simulink model "MMC_phase_discentralized_HAAS_20260927"  (R2024b)
settings: Solver=FixedStepDiscrete  StartTime=t_init_sim  StopTime=sim_time  FixedStep=Ts  RelTol=1e-3
values from neighbouring files (symbols this model uses):
  a = 1    [script_MMC_phase_hackathon_NLM_discentralized_HAAS_20260927.m]
  C1low1_active = 1    [script_MMC_phase_hackathon_NLM_discentralized_HAAS_20260927.m]
  C2low1_active = 1    [script_MMC_phase_hackathon_NLM_discentralized_HAAS_20260927.m]
  C_bus = 4400e-6    (= 0.0044)    [script_MMC_phase_hackathon_NLM_discentralized_HAAS_20260927.m]
  C_M_extra = C_m-twist_high_side_C    [script_MMC_phase_hackathon_NLM_discentralized_HAAS_20260927.m]
  duty_cycle = 1.0    (= 1)    [script_MMC_phase_hackathon_NLM_discentralized_HAAS_20260927.m]
  f0 = 50    [script_MMC_phase_hackathon_NLM_discentralized_HAAS_20260927.m]
  feeder_current_lower_rate_limit = -10    [script_MMC_phase_hackathon_NLM_discentralized_HAAS_20260927.m]    (also in twist_parameters.m = -500)
  feeder_current_tab = [0.328 0.217 0.162 0.132 0.109 0.094 0.083 0.075 0.068 0.062 0.058 0.054 ... (42 elements, 14x3)]    [feeder_current.mat]
  feeder_current_upper_rate_limit = 0.386/(20e-3)    (= 19.3)    [twist_parameters.m]
  is6VExternallySupplied = true    [script_MMC_phase_hackathon_NLM_discentralized_HAAS_20260927.m]
  isFeederJumperOpen = true    [script_MMC_phase_hackathon_NLM_discentralized_HAAS_20260927.m]
  L_arm = 30e-3    (= 0.03)    [script_MMC_phase_hackathon_NLM_discentralized_HAAS_20260927.m]
  m = 1    [script_MMC_phase_hackathon_NLM_discentralized_HAAS_20260927.m]
  N = 5    [script_MMC_phase_hackathon_NLM_discentralized_HAAS_20260927.m]
  power_losses = false    [script_MMC_phase_hackathon_NLM_discentralized_HAAS_20260927.m]
  R = 15    [script_MMC_phase_hackathon_NLM_discentralized_HAAS_20260927.m]
  R_arm = 0.2    [script_MMC_phase_hackathon_NLM_discentralized_HAAS_20260927.m]
  source_V = 0    [script_MMC_phase_hackathon_NLM_discentralized_HAAS_20260927.m]
  Tcom_sample = round(Tcom / Ts)    [script_MMC_phase_hackathon_NLM_discentralized_HAAS_20260927.m]
  time_charge = 0.1    [script_MMC_phase_hackathon_NLM_discentralized_HAAS_20260927.m]
  time_decharge = 1.5    [script_MMC_phase_hackathon_NLM_discentralized_HAAS_20260927.m]
  Ts = 1e-6    (= 1e-06)    [script_MMC_phase_hackathon_NLM_discentralized_HAAS_20260927.m]
  twist_data_acquisition_delay = 50e-9    (= 5e-08)    [script_MMC_phase_hackathon_NLM_discentralized_HAAS_20260927.m]    (also in twist_parameters.m)
  twist_data_sampling_period = 1/twist_freq_data_sampling    (= 5e-05)    [script_MMC_phase_hackathon_NLM_discentralized_HAAS_20260927.m]    (also in twist_parameters.m)
  twist_dead_time = 200e-9    (= 2e-07)    [twist_parameters.m]
  twist_freq_switching = 200e3    (= 200000)    [twist_parameters.m]
  twist_high_side_adc_R = 1/(1/2e6 + 1/2e6 + 1/(330e3+5.6e3))    (= 251272.836178)    [twist_parameters.m]
  twist_high_side_C = 33e-6*4 + 4.7e-6*12    (= 0.0001884)    [twist_parameters.m]
  twist_high_side_feeder_R = 47e3+4.7e3    (= 51700)    [twist_parameters.m]
  twist_high_side_rC = 0.1    [twist_parameters.m]
  twist_low_side_adc_R = 150e3+470    (= 150470)    [twist_parameters.m]
  twist_low_side_C_ceramic = 3*4.7e-6    (= 1.41e-05)    [twist_parameters.m]
  twist_low_side_C_electrolytic = 47e-6    (= 4.7e-05)    [twist_parameters.m]
  twist_low_side_L = 33e-6    (= 3.3e-05)    [twist_parameters.m]
  twist_low_side_rC = 700e-3    (= 0.7)    [twist_parameters.m]
  twist_low_side_rL = 20e-3    (= 0.02)    [twist_parameters.m]
  twist_R_VCC = (tau_VCC/twist_high_side_C  - twist_high_side_rC)/(1-(tau_VCC/twist_high_side_C - twist_high_side_rC)/R_parallel)    (= 1110.74997822)    [twist_parameters.m]
  VDC = 48    [script_MMC_phase_hackathon_NLM_discentralized_HAAS_20260927.m]
undefined symbols (not defined in the file or in its folder): C_SM, feeder_current, gcbh, sps_rtmsupport, twist_low_side_lC
libraries: spsSeriesRLCBranchLib x135, spsTriangleGeneratorLib x60, spsMosfetLib x60, spsCurrentMeasurementLib x43, spsVoltageMeasurementLib x35, spsControlledCurrentSourceLib x30, spsDiodeLib x22, spsIdealSwitchLib x20, spsControlledVoltageSourceLib x1, spsGroundLib x1, spspowerguiLib x1
(part 4 of 22)

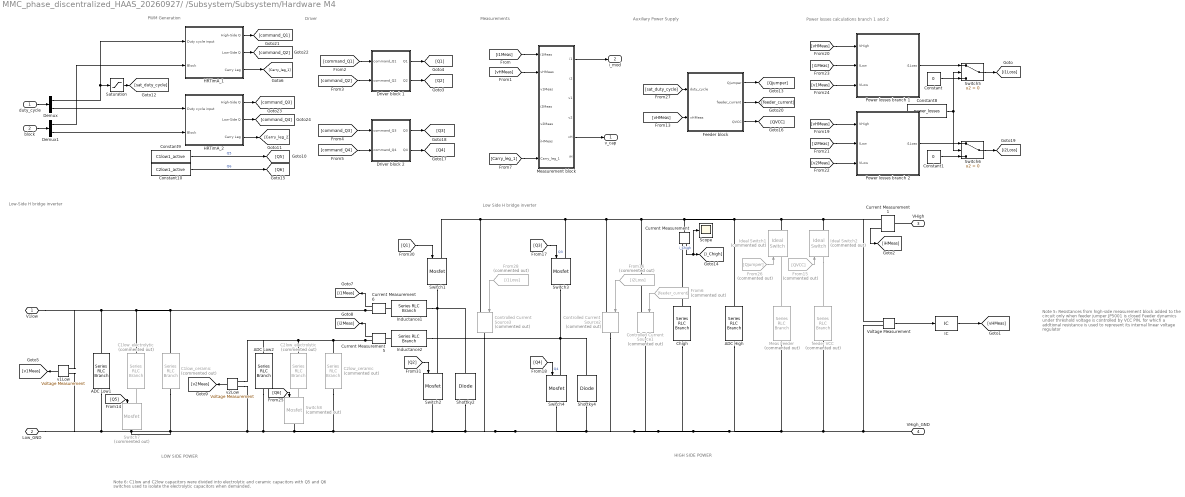
== system MMC_phase_discentralized_HAAS_20260927/ /Subsystem/Subsystem/Hardware M4 ==
  note: Low Side H bridge inverter
  note: PWM Generation
  note: Auxiliary Power Supply
  note: LOW SIDE POWER
  note: Low-Side H bridge inverter
  note: Power losses calculations branch 1 and 2
  note: Note 6:
      | C1low and C2low capacitors were divided into electrolytic and ceramic capacitors with Q5 and Q6 switches used to isolate the electrolytic capacitors when demanded.
  note: HIGH SIDE POWER
  note: Measurements
  note: Note 5:
      |
      | Resistances from high-side measurement block added to the circuit only when feeder jumper JP5001 is closed
      |
      | Feeder dynamics under threshold voltage is controlled by VCC PIN, for which a addtional resistance is used to represent its internal linear voltage regulator
  note: Driver
  duty_cycle : Inport
  block : Inport  Port=2
  ADC High : spsSeriesRLCBranchLib/Series RLC Branch  LConnTagsString=__new0  RConnTagsString=__new0  BranchType=R  Resistance=twist_high_side_adc_R  Inductance=twist_low_side_L  SetiL0=off  InitialCurrent=0  Capacitance=1e-6  Setx0=off  InitialVoltage=0  Measurements=None
  ADC Low1 : spsSeriesRLCBranchLib/Series RLC Branch  LConnTagsString=__new0  RConnTagsString=__new0  BranchType=R  Resistance=twist_low_side_adc_R  Inductance=twist_low_side_L  SetiL0=off  InitialCurrent=0  Capacitance=1e-6  Setx0=off  InitialVoltage=0  Measurements=Branch voltage
  ADC Low2 : spsSeriesRLCBranchLib/Series RLC Branch  LConnTagsString=__new0  RConnTagsString=__new0  BranchType=R  Resistance=twist_low_side_adc_R  Inductance=twist_low_side_L  SetiL0=off  InitialCurrent=0  Capacitance=1e-6  Setx0=off  InitialVoltage=0  Measurements=Branch voltage
  C1low_ceramic : spsSeriesRLCBranchLib/Series RLC Branch  Commented=on  LConnTagsString=__new0  RConnTagsString=__new0  BranchType=C  Resistance=twist_low_side_rC  Inductance=1e-3  SetiL0=off  InitialCurrent=0  Capacitance=twist_low_side_C_ceramic  Setx0=off  InitialVoltage=source_V  Measurements=None
  C1low_electrolytic : spsSeriesRLCBranchLib/Series RLC Branch  Commented=on  LConnTagsString=__new0  RConnTagsString=__new0  BranchType=RC  Resistance=twist_low_side_rC  Inductance=twist_low_side_lC  SetiL0=off  InitialCurrent=0  Capacitance=twist_low_side_C_electrolytic  Setx0=off  InitialVoltage=source_V  Measurements=None
  C2low_ceramic : spsSeriesRLCBranchLib/Series RLC Branch  Commented=on  LConnTagsString=__new0  RConnTagsString=__new0  BranchType=C  Resistance=twist_low_side_rC  Inductance=1e-3  SetiL0=off  InitialCurrent=0  Capacitance=twist_low_side_C_ceramic  Setx0=off  InitialVoltage=source_V  Measurements=None
  C2low_electrolytic : spsSeriesRLCBranchLib/Series RLC Branch  Commented=on  LConnTagsString=__new0  RConnTagsString=__new0  BranchType=RC  Resistance=twist_low_side_rC  Inductance=twist_low_side_lC  SetiL0=off  InitialCurrent=0  Capacitance=twist_low_side_C_electrolytic  Setx0=off  InitialVoltage=source_V  Measurements=None
  Chigh : spsSeriesRLCBranchLib/Series RLC Branch  LConnTagsString=__new0  RConnTagsString=__new0  BranchType=RC  Resistance=twist_high_side_rC  Inductance=1e-3  SetiL0=off  InitialCurrent=0  Capacitance=twist_high_side_C  Setx0=on  InitialVoltage=source_V  Measurements=None
  Constant : Constant  Value=0
  Constant1 : Constant  Value=0
  Constant10 : Constant  Value=C2low1_active
  Constant8 : Constant  Value=power_losses
  Constant9 : Constant  Value=C1low1_active
  Controlled Current Source1 : spsControlledCurrentSourceLib/Controlled Current Source  Commented=on  Initialize=on  Source_Type=AC  Amplitude=0  Phase=0  Frequency=0  Measurements=None
  Controlled Current Source2 : spsControlledCurrentSourceLib/Controlled Current Source  Commented=on  Initialize=on  Source_Type=AC  Amplitude=0  Phase=0  Frequency=0  Measurements=None
  Controlled Current Source3 : spsControlledCurrentSourceLib/Controlled Current Source  Commented=on  Initialize=on  Source_Type=AC  Amplitude=0  Phase=0  Frequency=0  Measurements=None
  Current Measurement{,1,5..6} (4 alike) : spsCurrentMeasurementLib/Current Measurement  PhasorSimulation=off  OutputType=Complex  PSBequivalent=0
  Demux : Demux  Outputs=2
  Demux1 : Demux  Outputs=2
  Driver block 1 : Subsystem
  Driver block 2 : Subsystem
  Feeder block : Subsystem
  From15 : From  Commented=on  GotoTag=QVCC
  From16 : From  Commented=on  GotoTag=i2Loss
  From26 : From  Commented=on  GotoTag=Qjumper
  From28 : From  Commented=on  GotoTag=i1Loss
  From6 : From  Commented=on  GotoTag=feeder_current
  HRTimA_1 : Subsystem
  HRTimA_2 : Subsystem
  IC : InitialCondition  Value=source_V
  Ideal Switch1 : spsIdealSwitchLib/Ideal Switch  Commented=on  Ron=0.001  Lon=0  IC=0  Rs=1e5  Cs=inf  Measurements=on
  Ideal Switch2 : spsIdealSwitchLib/Ideal Switch  Commented=on  Ron=0.001  Lon=0  IC=0  Rs=1e5  Cs=inf  Measurements=on
  Inductance1 : spsSeriesRLCBranchLib/Series RLC Branch  LConnTagsString=__new0  RConnTagsString=__new0  BranchType=RL  Resistance=twist_low_side_rL  Inductance=twist_low_side_L  SetiL0=off  InitialCurrent=0  Capacitance=1e-6  Setx0=off  InitialVoltage=0  Measurements=None
  Inductance2 : spsSeriesRLCBranchLib/Series RLC Branch  LConnTagsString=__new0  RConnTagsString=__new0  BranchType=RL  Resistance=twist_low_side_rL  Inductance=twist_low_side_L  SetiL0=off  InitialCurrent=0  Capacitance=1e-6  Setx0=off  InitialVoltage=0  Measurements=None
  Meas Feeder : spsSeriesRLCBranchLib/Series RLC Branch  Commented=on  LConnTagsString=__new0  RConnTagsString=__new0  BranchType=R  Resistance=twist_high_side_feeder_R  Inductance=twist_low_side_L  SetiL0=off  InitialCurrent=0  Capacitance=1e-6  Setx0=off  InitialVoltage=0  Measurements=None
  Measurement block : Subsystem
  Power losses branch 1 : Subsystem
  Power losses branch 2 : Subsystem
  Saturation : Saturate  UpperLimit=1  LowerLimit=0
  Scope : Scope
  Shottky2 : spsDiodeLib/Diode  Ron=twist_shottky_Ron  Lon=0  Vf=twist_shottky_Vf  IC=0  UseSnubber=0  Rs=twist_shottky_Rs  Cs=twist_shottky_Cs  Measurements=off
  Shottky4 : spsDiodeLib/Diode  Ron=twist_shottky_Ron  Lon=0  Vf=twist_shottky_Vf  IC=0  UseSnubber=0  Rs=twist_shottky_Rs  Cs=twist_shottky_Cs  Measurements=off
  Switch{1..4} (4 alike) : spsMosfetLib/Mosfet  Ron=twist_FET_Ron  Lon=0  Rd=twist_FET_Rd  Vfd=twist_FET_Vf  IC=0  Rs=twist_FET_Rs  Cs=twist_FET_Cs  Measurements=off
  Switch5 : Switch  Criteria=u2 > Threshold  SaturateOnIntegerOverflow=off  InputSameDT=off
  Switch6 : Switch  Criteria=u2 > Threshold  SaturateOnIntegerOverflow=off  InputSameDT=off
  Switch7 : spsMosfetLib/Mosfet  Commented=on  Ron=twist_FET_Clow_Ron  Lon=0  Rd=twist_FET_Clow_Ron  Vfd=0  IC=0  Rs=twist_FET_Rs  Cs=twist_FET_Cs  Measurements=off
  Switch8 : spsMosfetLib/Mosfet  Commented=on  Ron=twist_FET_Clow_Ron  Lon=0  Rd=twist_FET_Clow_Ron  Vfd=0  IC=0  Rs=twist_FET_Rs  Cs=twist_FET_Cs  Measurements=off
  Voltage Measurement : spsVoltageMeasurementLib/Voltage Measurement  PhasorSimulation=off  OutputType=Complex  PSBequivalent=0
  feeder VCC : spsSeriesRLCBranchLib/Series RLC Branch  Commented=on  LConnTagsString=__new0  RConnTagsString=__new0  BranchType=R  Resistance=twist_R_VCC  Inductance=twist_low_side_L  SetiL0=off  InitialCurrent=0  Capacitance=1e-6  Setx0=off  InitialVoltage=0  Measurements=None
  v1Low : spsVoltageMeasurementLib/Voltage Measurement  PhasorSimulation=off  OutputType=Complex  PSBequivalent=0
  v2Low : spsVoltageMeasurementLib/Voltage Measurement  PhasorSimulation=off  OutputType=Complex  PSBequivalent=0
  V1low : PMIOPort  Side=Left
  Low_GND : PMIOPort  Port=2  Side=Left
  VHigh : PMIOPort  Port=3  Side=Right
  VHigh_GND : PMIOPort  Port=4  Side=Right
  v_cap : Outport
  i_mod : Outport  Port=2
  wires:
  Constant8/1 -> Switch5/2, Switch6/2
  Constant9/1 -> [Q5]  "Q5"
  Constant1/1 -> Switch6/3
  v1Low/1 -> [v1Meas]
  Power losses branch 1/1(i1Loss) -> Switch5/1
  Constant/1 -> Switch5/3
  [Q1] -> Switch1/1
  [Q3] -> Switch3/1  "Q3"
  Voltage Measurement/1 -> IC/1
  Constant10/1 -> [Q6]  "Q6"
  [v1Meas] -> Power losses branch 1/3(VLow)
  [i2Meas] -> Power losses branch 2/2(ILow)
  Switch5/1 -> [i1Loss]
  HRTimA_2/3(Carry Leg) -> [Carry_leg_2]
  Current Measurement1/1 -> [iHMeas]
  v2Low/1 -> [v2Meas]
  HRTimA_1/3(Carry Leg) -> [Carry_leg_1]
  [vHMeas] -> Power losses branch 1/1(VHigh)
  IC/1 -> [vHMeas]
  From28/1 -> Controlled Current Source3/1
  Current Measurement/1 -> Scope/1, [i_Chigh]  "i_Chigh"
  Switch6/1 -> [i2Loss]
  Current Measurement5/1 -> [i2Meas]
  From26/1 -> Ideal Switch1/1
  [i1Meas] -> Power losses branch 1/2(ILow)
  From15/1 -> Ideal Switch2/1
  [Q5] -> Switch7/1
  [Q6] -> Switch8/1
  [Q4] -> Switch4/1  "Q4"
  [Q2] -> Switch2/1
  From6/1 -> Controlled Current Source1/1
  [vHMeas] -> Power losses branch 2/1(VHigh)
  From16/1 -> Controlled Current Source2/1
  [v2Meas] -> Power losses branch 2/3(VLow)
  Current Measurement6/1 -> [i1Meas]
  Power losses branch 2/1(i1Loss) -> Switch6/1
  duty_cycle/1 -> Demux/1
  Demux/1 -> Saturation/1, HRTimA_1/1(Duty cycle input)
  Demux1/1 -> HRTimA_1/2(Block)
  block/1 -> Demux1/1
  Demux1/2 -> HRTimA_2/2(Block)
  Demux/2 -> HRTimA_2/1(Duty cycle input)
  [vHMeas] -> Feeder block/2(vHMeas)
  Saturation/1 -> [sat_duty_cycle]
  [sat_duty_cycle] -> Feeder block/1(duty_cycle)
  Feeder block/1(Qjumper) -> [Qjumper]
  Feeder block/3(QVCC) -> [QVCC]
  Feeder block/2(feeder_current) -> [feeder_current]
  Measurement block/1(i1) -> i_mod/1
  [i1Meas] -> Measurement block/1(i1Meas)
  [vHMeas] -> Measurement block/2(vHMeas)
  Measurement block/5(vH) -> v_cap/1
  HRTimA_1/1(High-Side Q) -> [command_Q1]
  HRTimA_1/2(Low-Side Q) -> [command_Q2]
  HRTimA_2/1(High-Side Q) -> [command_Q3]
  HRTimA_2/2(Low-Side Q) -> [command_Q4]
  [command_Q1] -> Driver block 1/1(command_Q1)
  [command_Q2] -> Driver block 1/2(command_Q2)
  [command_Q3] -> Driver block 2/1(command_Q3)
  [command_Q4] -> Driver block 2/2(command_Q4)
  Driver block 1/1(Q1) -> [Q1]
  Driver block 1/2(Q2) -> [Q2]
  Driver block 2/1(Q3) -> [Q3]
  Driver block 2/2(Q4) -> [Q4]
  [Carry_leg_1] -> Measurement block/7(Carry_leg_1)
  connections:
  Current Measurement6/RConn1 -- v1Low/LConn1 -- V1low/RConn1 -- ADC Low1/LConn1 -- C1low_electrolytic/LConn1 -- C1low_ceramic/LConn1
  Switch3/LConn1 -- Controlled Current Source3/LConn1 -- Switch1/LConn1 -- Current Measurement/LConn1 -- Ideal Switch1/RConn1 -- Voltage Measurement/LConn1 -- Current Measurement1/RConn1 -- Ideal Switch2/RConn1 -- ADC High/LConn1 -- Controlled Current Source1/LConn1 -- Controlled Current Source2/LConn1
  VHigh_GND/RConn1 -- Voltage Measurement/LConn2 -- feeder VCC/RConn1 -- ADC High/RConn1 -- Chigh/RConn1 -- Controlled Current Source2/RConn1 -- Controlled Current Source3/RConn1 -- Switch2/RConn1 -- Low_GND/RConn1 -- v1Low/LConn2 -- ADC Low1/RConn1 -- Switch7/RConn1 -- C1low_ceramic/RConn1 -- v2Low/LConn2 -- ADC Low2/RConn1 -- Switch8/RConn1 -- C2low_ceramic/RConn1 -- Shottky2/LConn1 -- Switch4/RConn1 -- Shottky4/LConn1 -- Controlled Current Source1/RConn1 -- Meas Feeder/RConn1
  Current Measurement5/RConn1 -- v2Low/LConn1 -- ADC Low2/LConn1 -- C2low_electrolytic/LConn1 -- C2low_ceramic/LConn1
  Inductance2/RConn1 -- Switch4/LConn1 -- Switch3/RConn1 -- Shottky4/RConn1
  Switch1/RConn1 -- Inductance1/RConn1 -- Shottky2/RConn1 -- Switch2/LConn1
  Meas Feeder/LConn1 -- Ideal Switch1/LConn1
  Inductance2/LConn1 -- Current Measurement5/LConn1
  Switch7/LConn1 -- C1low_electrolytic/RConn1
  Ideal Switch2/LConn1 -- feeder VCC/LConn1
  Switch8/LConn1 -- C2low_electrolytic/RConn1
  Current Measurement/RConn1 -- Chigh/LConn1
  VHigh/RConn1 -- Current Measurement1/LConn1
  Current Measurement6/LConn1 -- Inductance1/LConn1

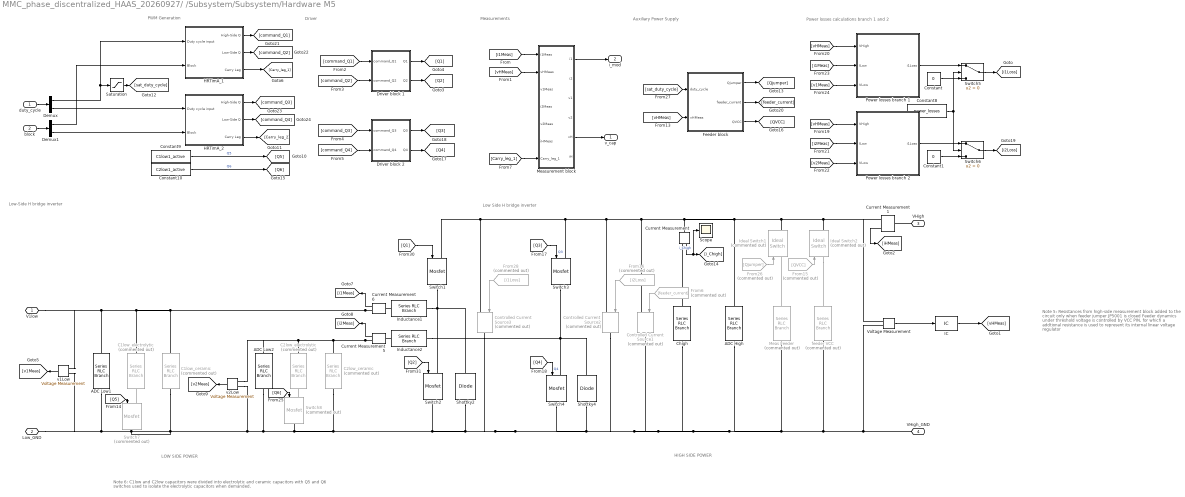
== system MMC_phase_discentralized_HAAS_20260927/ /Subsystem/Subsystem/Hardware M5 ==
  note: Low Side H bridge inverter
  note: PWM Generation
  note: Auxiliary Power Supply
  note: LOW SIDE POWER
  note: Low-Side H bridge inverter
  note: Power losses calculations branch 1 and 2
  note: Note 6:
      | C1low and C2low capacitors were divided into electrolytic and ceramic capacitors with Q5 and Q6 switches used to isolate the electrolytic capacitors when demanded.
  note: HIGH SIDE POWER
  note: Measurements
  note: Note 5:
      |
      | Resistances from high-side measurement block added to the circuit only when feeder jumper JP5001 is closed
      |
      | Feeder dynamics under threshold voltage is controlled by VCC PIN, for which a addtional resistance is used to represent its internal linear voltage regulator
  note: Driver
  duty_cycle : Inport
  block : Inport  Port=2
  ADC High : spsSeriesRLCBranchLib/Series RLC Branch  LConnTagsString=__new0  RConnTagsString=__new0  BranchType=R  Resistance=twist_high_side_adc_R  Inductance=twist_low_side_L  SetiL0=off  InitialCurrent=0  Capacitance=1e-6  Setx0=off  InitialVoltage=0  Measurements=None
  ADC Low1 : spsSeriesRLCBranchLib/Series RLC Branch  LConnTagsString=__new0  RConnTagsString=__new0  BranchType=R  Resistance=twist_low_side_adc_R  Inductance=twist_low_side_L  SetiL0=off  InitialCurrent=0  Capacitance=1e-6  Setx0=off  InitialVoltage=0  Measurements=Branch voltage
  ADC Low2 : spsSeriesRLCBranchLib/Series RLC Branch  LConnTagsString=__new0  RConnTagsString=__new0  BranchType=R  Resistance=twist_low_side_adc_R  Inductance=twist_low_side_L  SetiL0=off  InitialCurrent=0  Capacitance=1e-6  Setx0=off  InitialVoltage=0  Measurements=Branch voltage
  C1low_ceramic : spsSeriesRLCBranchLib/Series RLC Branch  Commented=on  LConnTagsString=__new0  RConnTagsString=__new0  BranchType=C  Resistance=twist_low_side_rC  Inductance=1e-3  SetiL0=off  InitialCurrent=0  Capacitance=twist_low_side_C_ceramic  Setx0=off  InitialVoltage=source_V  Measurements=None
  C1low_electrolytic : spsSeriesRLCBranchLib/Series RLC Branch  Commented=on  LConnTagsString=__new0  RConnTagsString=__new0  BranchType=RC  Resistance=twist_low_side_rC  Inductance=twist_low_side_lC  SetiL0=off  InitialCurrent=0  Capacitance=twist_low_side_C_electrolytic  Setx0=off  InitialVoltage=source_V  Measurements=None
  C2low_ceramic : spsSeriesRLCBranchLib/Series RLC Branch  Commented=on  LConnTagsString=__new0  RConnTagsString=__new0  BranchType=C  Resistance=twist_low_side_rC  Inductance=1e-3  SetiL0=off  InitialCurrent=0  Capacitance=twist_low_side_C_ceramic  Setx0=off  InitialVoltage=source_V  Measurements=None
  C2low_electrolytic : spsSeriesRLCBranchLib/Series RLC Branch  Commented=on  LConnTagsString=__new0  RConnTagsString=__new0  BranchType=RC  Resistance=twist_low_side_rC  Inductance=twist_low_side_lC  SetiL0=off  InitialCurrent=0  Capacitance=twist_low_side_C_electrolytic  Setx0=off  InitialVoltage=source_V  Measurements=None
  Chigh : spsSeriesRLCBranchLib/Series RLC Branch  LConnTagsString=__new0  RConnTagsString=__new0  BranchType=RC  Resistance=twist_high_side_rC  Inductance=1e-3  SetiL0=off  InitialCurrent=0  Capacitance=twist_high_side_C  Setx0=on  InitialVoltage=source_V  Measurements=None
  Constant : Constant  Value=0
  Constant1 : Constant  Value=0
  Constant10 : Constant  Value=C2low1_active
  Constant8 : Constant  Value=power_losses
  Constant9 : Constant  Value=C1low1_active
  Controlled Current Source1 : spsControlledCurrentSourceLib/Controlled Current Source  Commented=on  Initialize=on  Source_Type=AC  Amplitude=0  Phase=0  Frequency=0  Measurements=None
  Controlled Current Source2 : spsControlledCurrentSourceLib/Controlled Current Source  Commented=on  Initialize=on  Source_Type=AC  Amplitude=0  Phase=0  Frequency=0  Measurements=None
  Controlled Current Source3 : spsControlledCurrentSourceLib/Controlled Current Source  Commented=on  Initialize=on  Source_Type=AC  Amplitude=0  Phase=0  Frequency=0  Measurements=None
  Current Measurement{,1,5..6} (4 alike) : spsCurrentMeasurementLib/Current Measurement  PhasorSimulation=off  OutputType=Complex  PSBequivalent=0
  Demux : Demux  Outputs=2
  Demux1 : Demux  Outputs=2
  Driver block 1 : Subsystem
  Driver block 2 : Subsystem
  Feeder block : Subsystem
  From15 : From  Commented=on  GotoTag=QVCC
  From16 : From  Commented=on  GotoTag=i2Loss
  From26 : From  Commented=on  GotoTag=Qjumper
  From28 : From  Commented=on  GotoTag=i1Loss
  From6 : From  Commented=on  GotoTag=feeder_current
  HRTimA_1 : Subsystem
  HRTimA_2 : Subsystem
  IC : InitialCondition  Value=source_V
  Ideal Switch1 : spsIdealSwitchLib/Ideal Switch  Commented=on  Ron=0.001  Lon=0  IC=0  Rs=1e5  Cs=inf  Measurements=on
  Ideal Switch2 : spsIdealSwitchLib/Ideal Switch  Commented=on  Ron=0.001  Lon=0  IC=0  Rs=1e5  Cs=inf  Measurements=on
  Inductance1 : spsSeriesRLCBranchLib/Series RLC Branch  LConnTagsString=__new0  RConnTagsString=__new0  BranchType=RL  Resistance=twist_low_side_rL  Inductance=twist_low_side_L  SetiL0=off  InitialCurrent=0  Capacitance=1e-6  Setx0=off  InitialVoltage=0  Measurements=None
  Inductance2 : spsSeriesRLCBranchLib/Series RLC Branch  LConnTagsString=__new0  RConnTagsString=__new0  BranchType=RL  Resistance=twist_low_side_rL  Inductance=twist_low_side_L  SetiL0=off  InitialCurrent=0  Capacitance=1e-6  Setx0=off  InitialVoltage=0  Measurements=None
  Meas Feeder : spsSeriesRLCBranchLib/Series RLC Branch  Commented=on  LConnTagsString=__new0  RConnTagsString=__new0  BranchType=R  Resistance=twist_high_side_feeder_R  Inductance=twist_low_side_L  SetiL0=off  InitialCurrent=0  Capacitance=1e-6  Setx0=off  InitialVoltage=0  Measurements=None
  Measurement block : Subsystem
  Power losses branch 1 : Subsystem
  Power losses branch 2 : Subsystem
  Saturation : Saturate  UpperLimit=1  LowerLimit=0
  Scope : Scope
  Shottky2 : spsDiodeLib/Diode  Ron=twist_shottky_Ron  Lon=0  Vf=twist_shottky_Vf  IC=0  UseSnubber=0  Rs=twist_shottky_Rs  Cs=twist_shottky_Cs  Measurements=off
  Shottky4 : spsDiodeLib/Diode  Ron=twist_shottky_Ron  Lon=0  Vf=twist_shottky_Vf  IC=0  UseSnubber=0  Rs=twist_shottky_Rs  Cs=twist_shottky_Cs  Measurements=off
  Switch{1..4} (4 alike) : spsMosfetLib/Mosfet  Ron=twist_FET_Ron  Lon=0  Rd=twist_FET_Rd  Vfd=twist_FET_Vf  IC=0  Rs=twist_FET_Rs  Cs=twist_FET_Cs  Measurements=off
  Switch5 : Switch  Criteria=u2 > Threshold  SaturateOnIntegerOverflow=off  InputSameDT=off
  Switch6 : Switch  Criteria=u2 > Threshold  SaturateOnIntegerOverflow=off  InputSameDT=off
  Switch7 : spsMosfetLib/Mosfet  Commented=on  Ron=twist_FET_Clow_Ron  Lon=0  Rd=twist_FET_Clow_Ron  Vfd=0  IC=0  Rs=twist_FET_Rs  Cs=twist_FET_Cs  Measurements=off
  Switch8 : spsMosfetLib/Mosfet  Commented=on  Ron=twist_FET_Clow_Ron  Lon=0  Rd=twist_FET_Clow_Ron  Vfd=0  IC=0  Rs=twist_FET_Rs  Cs=twist_FET_Cs  Measurements=off
  Voltage Measurement : spsVoltageMeasurementLib/Voltage Measurement  PhasorSimulation=off  OutputType=Complex  PSBequivalent=0
  feeder VCC : spsSeriesRLCBranchLib/Series RLC Branch  Commented=on  LConnTagsString=__new0  RConnTagsString=__new0  BranchType=R  Resistance=twist_R_VCC  Inductance=twist_low_side_L  SetiL0=off  InitialCurrent=0  Capacitance=1e-6  Setx0=off  InitialVoltage=0  Measurements=None
  v1Low : spsVoltageMeasurementLib/Voltage Measurement  PhasorSimulation=off  OutputType=Complex  PSBequivalent=0
  v2Low : spsVoltageMeasurementLib/Voltage Measurement  PhasorSimulation=off  OutputType=Complex  PSBequivalent=0
  V1low : PMIOPort  Side=Left
  Low_GND : PMIOPort  Port=2  Side=Left
  VHigh : PMIOPort  Port=3  Side=Right
  VHigh_GND : PMIOPort  Port=4  Side=Right
  v_cap : Outport
  i_mod : Outport  Port=2
  wires:
  Constant8/1 -> Switch5/2, Switch6/2
  Constant9/1 -> [Q5]  "Q5"
  Constant1/1 -> Switch6/3
  v1Low/1 -> [v1Meas]
  Power losses branch 1/1(i1Loss) -> Switch5/1
  Constant/1 -> Switch5/3
  [Q1] -> Switch1/1
  [Q3] -> Switch3/1  "Q3"
  Voltage Measurement/1 -> IC/1
  Constant10/1 -> [Q6]  "Q6"
  [v1Meas] -> Power losses branch 1/3(VLow)
  [i2Meas] -> Power losses branch 2/2(ILow)
  Switch5/1 -> [i1Loss]
  HRTimA_2/3(Carry Leg) -> [Carry_leg_2]
  Current Measurement1/1 -> [iHMeas]
  v2Low/1 -> [v2Meas]
  HRTimA_1/3(Carry Leg) -> [Carry_leg_1]
  [vHMeas] -> Power losses branch 1/1(VHigh)
  IC/1 -> [vHMeas]
  From28/1 -> Controlled Current Source3/1
  Current Measurement/1 -> Scope/1, [i_Chigh]  "i_Chigh"
  Switch6/1 -> [i2Loss]
  Current Measurement5/1 -> [i2Meas]
  From26/1 -> Ideal Switch1/1
  [i1Meas] -> Power losses branch 1/2(ILow)
  From15/1 -> Ideal Switch2/1
  [Q5] -> Switch7/1
  [Q6] -> Switch8/1
  [Q4] -> Switch4/1  "Q4"
  [Q2] -> Switch2/1
  From6/1 -> Controlled Current Source1/1
  [vHMeas] -> Power losses branch 2/1(VHigh)
  From16/1 -> Controlled Current Source2/1
  [v2Meas] -> Power losses branch 2/3(VLow)
  Current Measurement6/1 -> [i1Meas]
  Power losses branch 2/1(i1Loss) -> Switch6/1
  duty_cycle/1 -> Demux/1
  Demux/1 -> Saturation/1, HRTimA_1/1(Duty cycle input)
  Demux1/1 -> HRTimA_1/2(Block)
  block/1 -> Demux1/1
  Demux1/2 -> HRTimA_2/2(Block)
  Demux/2 -> HRTimA_2/1(Duty cycle input)
  [vHMeas] -> Feeder block/2(vHMeas)
  Saturation/1 -> [sat_duty_cycle]
  [sat_duty_cycle] -> Feeder block/1(duty_cycle)
  Feeder block/1(Qjumper) -> [Qjumper]
  Feeder block/3(QVCC) -> [QVCC]
  Feeder block/2(feeder_current) -> [feeder_current]
  Measurement block/1(i1) -> i_mod/1
  [i1Meas] -> Measurement block/1(i1Meas)
  [vHMeas] -> Measurement block/2(vHMeas)
  Measurement block/5(vH) -> v_cap/1
  HRTimA_1/1(High-Side Q) -> [command_Q1]
  HRTimA_1/2(Low-Side Q) -> [command_Q2]
  HRTimA_2/1(High-Side Q) -> [command_Q3]
  HRTimA_2/2(Low-Side Q) -> [command_Q4]
  [command_Q1] -> Driver block 1/1(command_Q1)
  [command_Q2] -> Driver block 1/2(command_Q2)
  [command_Q3] -> Driver block 2/1(command_Q3)
  [command_Q4] -> Driver block 2/2(command_Q4)
  Driver block 1/1(Q1) -> [Q1]
  Driver block 1/2(Q2) -> [Q2]
  Driver block 2/1(Q3) -> [Q3]
  Driver block 2/2(Q4) -> [Q4]
  [Carry_leg_1] -> Measurement block/7(Carry_leg_1)
  connections:
  Current Measurement6/RConn1 -- v1Low/LConn1 -- V1low/RConn1 -- ADC Low1/LConn1 -- C1low_electrolytic/LConn1 -- C1low_ceramic/LConn1
  Switch3/LConn1 -- Controlled Current Source3/LConn1 -- Switch1/LConn1 -- Current Measurement/LConn1 -- Ideal Switch1/RConn1 -- Voltage Measurement/LConn1 -- Current Measurement1/RConn1 -- Ideal Switch2/RConn1 -- ADC High/LConn1 -- Controlled Current Source1/LConn1 -- Controlled Current Source2/LConn1
  VHigh_GND/RConn1 -- Voltage Measurement/LConn2 -- feeder VCC/RConn1 -- ADC High/RConn1 -- Chigh/RConn1 -- Controlled Current Source2/RConn1 -- Controlled Current Source3/RConn1 -- Switch2/RConn1 -- Low_GND/RConn1 -- v1Low/LConn2 -- ADC Low1/RConn1 -- Switch7/RConn1 -- C1low_ceramic/RConn1 -- v2Low/LConn2 -- ADC Low2/RConn1 -- Switch8/RConn1 -- C2low_ceramic/RConn1 -- Shottky2/LConn1 -- Switch4/RConn1 -- Shottky4/LConn1 -- Controlled Current Source1/RConn1 -- Meas Feeder/RConn1
  Current Measurement5/RConn1 -- v2Low/LConn1 -- ADC Low2/LConn1 -- C2low_electrolytic/LConn1 -- C2low_ceramic/LConn1
  Inductance2/RConn1 -- Switch4/LConn1 -- Switch3/RConn1 -- Shottky4/RConn1
  Switch1/RConn1 -- Inductance1/RConn1 -- Shottky2/RConn1 -- Switch2/LConn1
  Meas Feeder/LConn1 -- Ideal Switch1/LConn1
  Inductance2/LConn1 -- Current Measurement5/LConn1
  Switch7/LConn1 -- C1low_electrolytic/RConn1
  Ideal Switch2/LConn1 -- feeder VCC/LConn1
  Switch8/LConn1 -- C2low_electrolytic/RConn1
  Current Measurement/RConn1 -- Chigh/LConn1
  VHigh/RConn1 -- Current Measurement1/LConn1
  Current Measurement6/LConn1 -- Inductance1/LConn1

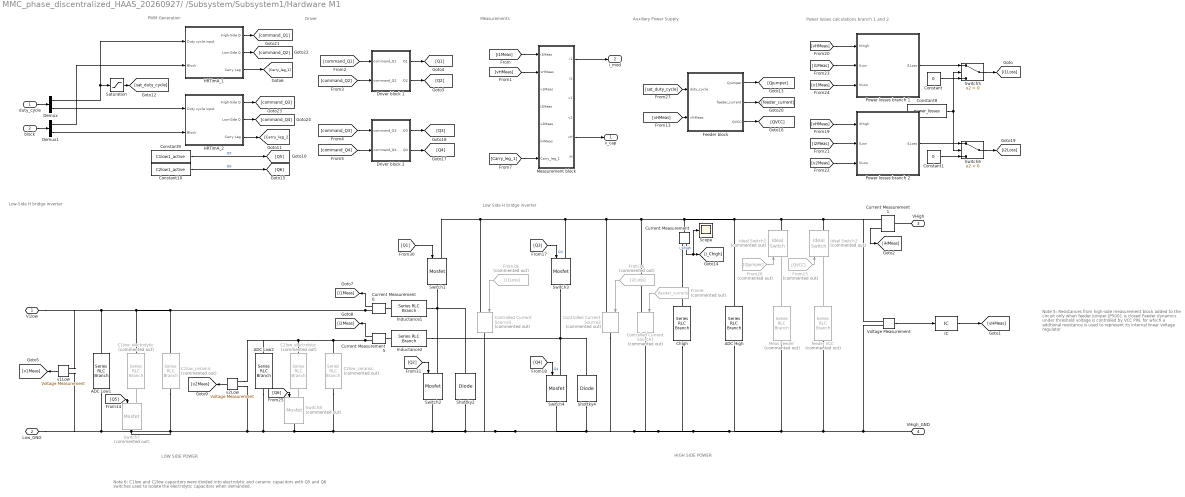
== system MMC_phase_discentralized_HAAS_20260927/ /Subsystem/Subsystem1/Hardware M1 ==
  note: Low Side H bridge inverter
  note: PWM Generation
  note: Auxiliary Power Supply
  note: LOW SIDE POWER
  note: Low-Side H bridge inverter
  note: Power losses calculations branch 1 and 2
  note: Note 6:
      | C1low and C2low capacitors were divided into electrolytic and ceramic capacitors with Q5 and Q6 switches used to isolate the electrolytic capacitors when demanded.
  note: HIGH SIDE POWER
  note: Measurements
  note: Note 5:
      |
      | Resistances from high-side measurement block added to the circuit only when feeder jumper JP5001 is closed
      |
      | Feeder dynamics under threshold voltage is controlled by VCC PIN, for which a addtional resistance is used to represent its internal linear voltage regulator
  note: Driver
  duty_cycle : Inport
  block : Inport  Port=2
  ADC High : spsSeriesRLCBranchLib/Series RLC Branch  LConnTagsString=__new0  RConnTagsString=__new0  BranchType=R  Resistance=twist_high_side_adc_R  Inductance=twist_low_side_L  SetiL0=off  InitialCurrent=0  Capacitance=1e-6  Setx0=off  InitialVoltage=0  Measurements=None
  ADC Low1 : spsSeriesRLCBranchLib/Series RLC Branch  LConnTagsString=__new0  RConnTagsString=__new0  BranchType=R  Resistance=twist_low_side_adc_R  Inductance=twist_low_side_L  SetiL0=off  InitialCurrent=0  Capacitance=1e-6  Setx0=off  InitialVoltage=0  Measurements=Branch voltage
  ADC Low2 : spsSeriesRLCBranchLib/Series RLC Branch  LConnTagsString=__new0  RConnTagsString=__new0  BranchType=R  Resistance=twist_low_side_adc_R  Inductance=twist_low_side_L  SetiL0=off  InitialCurrent=0  Capacitance=1e-6  Setx0=off  InitialVoltage=0  Measurements=Branch voltage
  C1low_ceramic : spsSeriesRLCBranchLib/Series RLC Branch  Commented=on  LConnTagsString=__new0  RConnTagsString=__new0  BranchType=C  Resistance=twist_low_side_rC  Inductance=1e-3  SetiL0=off  InitialCurrent=0  Capacitance=twist_low_side_C_ceramic  Setx0=off  InitialVoltage=source_V  Measurements=None
  C1low_electrolytic : spsSeriesRLCBranchLib/Series RLC Branch  Commented=on  LConnTagsString=__new0  RConnTagsString=__new0  BranchType=RC  Resistance=twist_low_side_rC  Inductance=twist_low_side_lC  SetiL0=off  InitialCurrent=0  Capacitance=twist_low_side_C_electrolytic  Setx0=off  InitialVoltage=source_V  Measurements=None
  C2low_ceramic : spsSeriesRLCBranchLib/Series RLC Branch  Commented=on  LConnTagsString=__new0  RConnTagsString=__new0  BranchType=C  Resistance=twist_low_side_rC  Inductance=1e-3  SetiL0=off  InitialCurrent=0  Capacitance=twist_low_side_C_ceramic  Setx0=off  InitialVoltage=source_V  Measurements=None
  C2low_electrolytic : spsSeriesRLCBranchLib/Series RLC Branch  Commented=on  LConnTagsString=__new0  RConnTagsString=__new0  BranchType=RC  Resistance=twist_low_side_rC  Inductance=twist_low_side_lC  SetiL0=off  InitialCurrent=0  Capacitance=twist_low_side_C_electrolytic  Setx0=off  InitialVoltage=source_V  Measurements=None
  Chigh : spsSeriesRLCBranchLib/Series RLC Branch  LConnTagsString=__new0  RConnTagsString=__new0  BranchType=RC  Resistance=twist_high_side_rC  Inductance=1e-3  SetiL0=off  InitialCurrent=0  Capacitance=twist_high_side_C  Setx0=on  InitialVoltage=source_V  Measurements=None
  Constant : Constant  Value=0
  Constant1 : Constant  Value=0
  Constant10 : Constant  Value=C2low1_active
  Constant8 : Constant  Value=power_losses
  Constant9 : Constant  Value=C1low1_active
  Controlled Current Source1 : spsControlledCurrentSourceLib/Controlled Current Source  Commented=on  Initialize=on  Source_Type=AC  Amplitude=0  Phase=0  Frequency=0  Measurements=None
  Controlled Current Source2 : spsControlledCurrentSourceLib/Controlled Current Source  Commented=on  Initialize=on  Source_Type=AC  Amplitude=0  Phase=0  Frequency=0  Measurements=None
  Controlled Current Source3 : spsControlledCurrentSourceLib/Controlled Current Source  Commented=on  Initialize=on  Source_Type=AC  Amplitude=0  Phase=0  Frequency=0  Measurements=None
  Current Measurement{,1,5..6} (4 alike) : spsCurrentMeasurementLib/Current Measurement  PhasorSimulation=off  OutputType=Complex  PSBequivalent=0
  Demux : Demux  Outputs=2
  Demux1 : Demux  Outputs=2
  Driver block 1 : Subsystem
  Driver block 2 : Subsystem
  Feeder block : Subsystem
  From15 : From  Commented=on  GotoTag=QVCC
  From16 : From  Commented=on  GotoTag=i2Loss
  From26 : From  Commented=on  GotoTag=Qjumper
  From28 : From  Commented=on  GotoTag=i1Loss
  From6 : From  Commented=on  GotoTag=feeder_current
  HRTimA_1 : Subsystem
  HRTimA_2 : Subsystem
  IC : InitialCondition  Value=source_V
  Ideal Switch1 : spsIdealSwitchLib/Ideal Switch  Commented=on  Ron=0.001  Lon=0  IC=0  Rs=1e5  Cs=inf  Measurements=on
  Ideal Switch2 : spsIdealSwitchLib/Ideal Switch  Commented=on  Ron=0.001  Lon=0  IC=0  Rs=1e5  Cs=inf  Measurements=on
  Inductance1 : spsSeriesRLCBranchLib/Series RLC Branch  LConnTagsString=__new0  RConnTagsString=__new0  BranchType=RL  Resistance=twist_low_side_rL  Inductance=twist_low_side_L  SetiL0=off  InitialCurrent=0  Capacitance=1e-6  Setx0=off  InitialVoltage=0  Measurements=None
  Inductance2 : spsSeriesRLCBranchLib/Series RLC Branch  LConnTagsString=__new0  RConnTagsString=__new0  BranchType=RL  Resistance=twist_low_side_rL  Inductance=twist_low_side_L  SetiL0=off  InitialCurrent=0  Capacitance=1e-6  Setx0=off  InitialVoltage=0  Measurements=None
  Meas Feeder : spsSeriesRLCBranchLib/Series RLC Branch  Commented=on  LConnTagsString=__new0  RConnTagsString=__new0  BranchType=R  Resistance=twist_high_side_feeder_R  Inductance=twist_low_side_L  SetiL0=off  InitialCurrent=0  Capacitance=1e-6  Setx0=off  InitialVoltage=0  Measurements=None
  Measurement block : Subsystem
  Power losses branch 1 : Subsystem
  Power losses branch 2 : Subsystem
  Saturation : Saturate  UpperLimit=1  LowerLimit=0
  Scope : Scope
  Shottky2 : spsDiodeLib/Diode  Ron=twist_shottky_Ron  Lon=0  Vf=twist_shottky_Vf  IC=0  UseSnubber=0  Rs=twist_shottky_Rs  Cs=twist_shottky_Cs  Measurements=off
  Shottky4 : spsDiodeLib/Diode  Ron=twist_shottky_Ron  Lon=0  Vf=twist_shottky_Vf  IC=0  UseSnubber=0  Rs=twist_shottky_Rs  Cs=twist_shottky_Cs  Measurements=off
  Switch{1..4} (4 alike) : spsMosfetLib/Mosfet  Ron=twist_FET_Ron  Lon=0  Rd=twist_FET_Rd  Vfd=twist_FET_Vf  IC=0  Rs=twist_FET_Rs  Cs=twist_FET_Cs  Measurements=off
  Switch5 : Switch  Criteria=u2 > Threshold  SaturateOnIntegerOverflow=off  InputSameDT=off
  Switch6 : Switch  Criteria=u2 > Threshold  SaturateOnIntegerOverflow=off  InputSameDT=off
  Switch7 : spsMosfetLib/Mosfet  Commented=on  Ron=twist_FET_Clow_Ron  Lon=0  Rd=twist_FET_Clow_Ron  Vfd=0  IC=0  Rs=twist_FET_Rs  Cs=twist_FET_Cs  Measurements=off
  Switch8 : spsMosfetLib/Mosfet  Commented=on  Ron=twist_FET_Clow_Ron  Lon=0  Rd=twist_FET_Clow_Ron  Vfd=0  IC=0  Rs=twist_FET_Rs  Cs=twist_FET_Cs  Measurements=off
  Voltage Measurement : spsVoltageMeasurementLib/Voltage Measurement  PhasorSimulation=off  OutputType=Complex  PSBequivalent=0
  feeder VCC : spsSeriesRLCBranchLib/Series RLC Branch  Commented=on  LConnTagsString=__new0  RConnTagsString=__new0  BranchType=R  Resistance=twist_R_VCC  Inductance=twist_low_side_L  SetiL0=off  InitialCurrent=0  Capacitance=1e-6  Setx0=off  InitialVoltage=0  Measurements=None
  v1Low : spsVoltageMeasurementLib/Voltage Measurement  PhasorSimulation=off  OutputType=Complex  PSBequivalent=0
  v2Low : spsVoltageMeasurementLib/Voltage Measurement  PhasorSimulation=off  OutputType=Complex  PSBequivalent=0
  V1low : PMIOPort  Side=Left
  Low_GND : PMIOPort  Port=2  Side=Left
  VHigh : PMIOPort  Port=3  Side=Right
  VHigh_GND : PMIOPort  Port=4  Side=Right
  v_cap : Outport
  i_mod : Outport  Port=2
  wires:
  Constant8/1 -> Switch5/2, Switch6/2
  Constant9/1 -> [Q5]  "Q5"
  Constant1/1 -> Switch6/3
  v1Low/1 -> [v1Meas]
  Power losses branch 1/1(i1Loss) -> Switch5/1
  Constant/1 -> Switch5/3
  [Q1] -> Switch1/1
  [Q3] -> Switch3/1  "Q3"
  Voltage Measurement/1 -> IC/1
  Constant10/1 -> [Q6]  "Q6"
  [v1Meas] -> Power losses branch 1/3(VLow)
  [i2Meas] -> Power losses branch 2/2(ILow)
  Switch5/1 -> [i1Loss]
  HRTimA_2/3(Carry Leg) -> [Carry_leg_2]
  Current Measurement1/1 -> [iHMeas]
  v2Low/1 -> [v2Meas]
  HRTimA_1/3(Carry Leg) -> [Carry_leg_1]
  [vHMeas] -> Power losses branch 1/1(VHigh)
  IC/1 -> [vHMeas]
  From28/1 -> Controlled Current Source3/1
  Current Measurement/1 -> Scope/1, [i_Chigh]  "i_Chigh"
  Switch6/1 -> [i2Loss]
  Current Measurement5/1 -> [i2Meas]
  From26/1 -> Ideal Switch1/1
  [i1Meas] -> Power losses branch 1/2(ILow)
  From15/1 -> Ideal Switch2/1
  [Q5] -> Switch7/1
  [Q6] -> Switch8/1
  [Q4] -> Switch4/1  "Q4"
  [Q2] -> Switch2/1
  From6/1 -> Controlled Current Source1/1
  [vHMeas] -> Power losses branch 2/1(VHigh)
  From16/1 -> Controlled Current Source2/1
  [v2Meas] -> Power losses branch 2/3(VLow)
  Current Measurement6/1 -> [i1Meas]
  Power losses branch 2/1(i1Loss) -> Switch6/1
  duty_cycle/1 -> Demux/1
  Demux/1 -> Saturation/1, HRTimA_1/1(Duty cycle input)
  Demux1/1 -> HRTimA_1/2(Block)
  block/1 -> Demux1/1
  Demux1/2 -> HRTimA_2/2(Block)
  Demux/2 -> HRTimA_2/1(Duty cycle input)
  [vHMeas] -> Feeder block/2(vHMeas)
  Saturation/1 -> [sat_duty_cycle]
  [sat_duty_cycle] -> Feeder block/1(duty_cycle)
  Feeder block/1(Qjumper) -> [Qjumper]
  Feeder block/3(QVCC) -> [QVCC]
  Feeder block/2(feeder_current) -> [feeder_current]
  Measurement block/1(i1) -> i_mod/1
  [i1Meas] -> Measurement block/1(i1Meas)
  [vHMeas] -> Measurement block/2(vHMeas)
  Measurement block/5(vH) -> v_cap/1
  HRTimA_1/1(High-Side Q) -> [command_Q1]
  HRTimA_1/2(Low-Side Q) -> [command_Q2]
  HRTimA_2/1(High-Side Q) -> [command_Q3]
  HRTimA_2/2(Low-Side Q) -> [command_Q4]
  [command_Q1] -> Driver block 1/1(command_Q1)
  [command_Q2] -> Driver block 1/2(command_Q2)
  [command_Q3] -> Driver block 2/1(command_Q3)
  [command_Q4] -> Driver block 2/2(command_Q4)
  Driver block 1/1(Q1) -> [Q1]
  Driver block 1/2(Q2) -> [Q2]
  Driver block 2/1(Q3) -> [Q3]
  Driver block 2/2(Q4) -> [Q4]
  [Carry_leg_1] -> Measurement block/7(Carry_leg_1)
  connections:
  Current Measurement6/RConn1 -- v1Low/LConn1 -- V1low/RConn1 -- ADC Low1/LConn1 -- C1low_electrolytic/LConn1 -- C1low_ceramic/LConn1
  Switch3/LConn1 -- Controlled Current Source3/LConn1 -- Switch1/LConn1 -- Current Measurement/LConn1 -- Ideal Switch1/RConn1 -- Voltage Measurement/LConn1 -- Current Measurement1/RConn1 -- Ideal Switch2/RConn1 -- ADC High/LConn1 -- Controlled Current Source1/LConn1 -- Controlled Current Source2/LConn1
  VHigh_GND/RConn1 -- Voltage Measurement/LConn2 -- feeder VCC/RConn1 -- ADC High/RConn1 -- Chigh/RConn1 -- Controlled Current Source2/RConn1 -- Controlled Current Source3/RConn1 -- Switch2/RConn1 -- Low_GND/RConn1 -- v1Low/LConn2 -- ADC Low1/RConn1 -- Switch7/RConn1 -- C1low_ceramic/RConn1 -- v2Low/LConn2 -- ADC Low2/RConn1 -- Switch8/RConn1 -- C2low_ceramic/RConn1 -- Shottky2/LConn1 -- Switch4/RConn1 -- Shottky4/LConn1 -- Controlled Current Source1/RConn1 -- Meas Feeder/RConn1
  Current Measurement5/RConn1 -- v2Low/LConn1 -- ADC Low2/LConn1 -- C2low_electrolytic/LConn1 -- C2low_ceramic/LConn1
  Inductance2/RConn1 -- Switch4/LConn1 -- Switch3/RConn1 -- Shottky4/RConn1
  Switch1/RConn1 -- Inductance1/RConn1 -- Shottky2/RConn1 -- Switch2/LConn1
  Meas Feeder/LConn1 -- Ideal Switch1/LConn1
  Inductance2/LConn1 -- Current Measurement5/LConn1
  Switch7/LConn1 -- C1low_electrolytic/RConn1
  Ideal Switch2/LConn1 -- feeder VCC/LConn1
  Switch8/LConn1 -- C2low_electrolytic/RConn1
  Current Measurement/RConn1 -- Chigh/LConn1
  VHigh/RConn1 -- Current Measurement1/LConn1
  Current Measurement6/LConn1 -- Inductance1/LConn1
